simulink model "EV"  (R2026b)
settings: Solver=VariableStepAuto
libraries: simulink x1
settings Model: Creator=Soundarya  LastModifiedBy=Soundarya

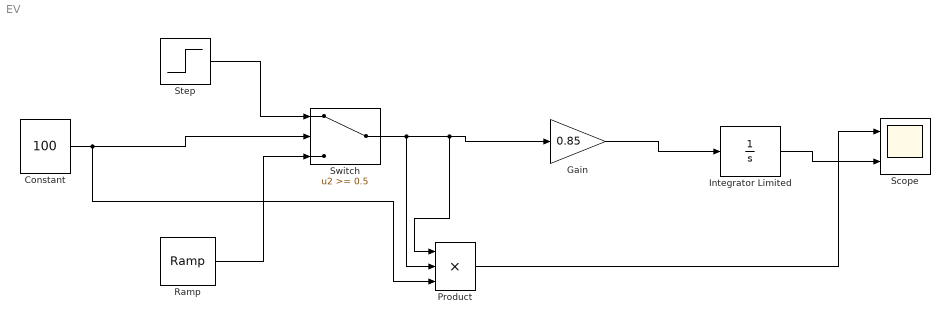
== system EV ==
  Constant : Constant  Value=100
  Gain : Gain  Gain=0.85
  Integrator Limited : Integrator  InitialCondition=50  LimitOutput=on  UpperSaturationLimit=100  LowerSaturationLimit=0
  Product : Product  Inputs=3
  Ramp : simulink/Sources/Ramp  slope=-16.2  start=5.0  InitialOutput=100.0
  Scope : Scope  NumInputPorts=2
      settings: ActiveDisplayYMinimum=-12.499999999999996  ActiveDisplayYMaximum=112.5
  Step : Step  Time=5  SampleTime=0
  Switch : Switch  Threshold=0.5  SaturateOnIntegerOverflow=off  InputSameDT=off
  wires:
  Step/1 -> Switch/1
  Constant/1 -> Product/3, Switch/2
  Ramp/1 -> Switch/3
  Switch/1 -> Product/2, Product/1, Gain/1
  Gain/1 -> Integrator Limited/1
  Product/1 -> Scope/1
  Integrator Limited/1 -> Scope/2
